simulink library "mssSimulink"  (R2024a)
settings: Solver=ode45  StartTime=0.0  StopTime=10.0  RelTol=1e-3
undefined symbols (not defined in the file): ABC, CN_data, CX_data, CY_data, D, G, Hoerner, K_supply, kt2ms, MA, magnitude, MRB, pathlength, RAO_Amp, RAO_Dir, RAO_Freq, RAO_Phase, RAO_Vel, RAO_yaw_back, RAO_yaw_quant, RAO_yaw_quantization_flag, rho_a, slcm, T_supply, table, vessel, vesselABC
libraries: $bdroot x99, simulink x13
(part 9 of 9)

== system mssSimulink/Environment/Wind/Wind/Wind gust/NORSOK spectrum ==
  Freqs : Inport
  u10 : Inport  Port=2
  5/(3n) (NORSOK parameter) : Constant  Value=5/(3*0.468)
  Constant2 : Constant
  Fcn2 : Fcn  Expr=u^(2/3)
  Fcn3 : Fcn  Expr=(u+1E-4)^(-3/4)
  Fcn4 : Fcn  Expr=u^0.45
  Gain1 : Gain  Gain=172  SaturateOnIntegerOverflow=on  OutDataTypeStr=Inherit: Same as input  ParamDataTypeStr=Inherit: Same as input
  Gain2 : Gain  Gain=1/10  SaturateOnIntegerOverflow=on  OutDataTypeStr=Inherit: Same as input  ParamDataTypeStr=Inherit: Same as input
  Gain3 : Gain  Gain=1/10  SaturateOnIntegerOverflow=on  OutDataTypeStr=Inherit: Same as input  ParamDataTypeStr=Inherit: Same as input
  Gain4 : Gain  Gain=320  SaturateOnIntegerOverflow=on  OutDataTypeStr=Inherit: Same as input  ParamDataTypeStr=Inherit: Same as input
  Math Function3 : Math  Operator=magnitude^2  SignedPower=on
  Math Function4 : Math  Operator=pow  SignedPower=on
  Math Function5 : Math  Operator=pow  SignedPower=on
  Product3 : Product  Inputs=3  SaturateOnIntegerOverflow=on  OutDataTypeStr=Inherit: Same as first input
  Product4 : Product  Inputs=/**  SaturateOnIntegerOverflow=on  OutDataTypeStr=Inherit: Same as first input
  Sum1 : Sum  Inputs=++|  SaturateOnIntegerOverflow=on
  n (NORSOK parameter) : Constant  Value=0.468
  z (height) : Constant  Value=Par_Wind_z
  S : Outport  VectorParamsAs1DForOutWhenUnconnected=off
  wires:
  Freqs/1 -> Gain1/1
  Gain1/1 -> Product3/1
  z (height)/1 -> Gain2/1
  Gain2/1 -> Fcn2/1, Fcn4/1
  Fcn2/1 -> Product3/2
  u10/1 -> Gain3/1
  Gain3/1 -> Fcn3/1, Math Function3/1
  Fcn3/1 -> Product3/3
  Product3/1 -> Math Function4/1  "x"
  n (NORSOK parameter)/1 -> Math Function4/2
  Math Function4/1 -> Sum1/2
  Constant2/1 -> Sum1/1
  Sum1/1 -> Math Function5/1
  Math Function5/1 -> Product4/1
  Fcn4/1 -> Gain4/1
  Math Function3/1 -> Product4/3
  Gain4/1 -> Product4/2
  Product4/1 -> S/1
  5/(3n) (NORSOK parameter)/1 -> Math Function5/2

== system mssSimulink/Environment/Wind/Wind/Wind gust/Phase generator ==
  Trigger : TriggerPort  VariantControl=(inherit)
  Random Number : RandomNumber  Variance=3  Seed=Par_Wind_phase_seed*[1:Par_Wind_nfreq]
  "SSA " : MATLABFcn  MATLABFcn=ssa
  Phase : Outport  VectorParamsAs1DForOutWhenUnconnected=off
  wires:
  Random Number/1 -> "SSA "/1
  "SSA "/1 -> Phase/1

== system mssSimulink/Hydrodynamics/Wave loads (U>0)/Wave loads U = U2/Wave loads for heading1/Wave component loop ==
  number of iterations : Inport
  Psi_r : Inport  Port=2
  Omega : Inport  Port=3
  Phase_tot : Inport  Port=4
  Zeta_a : Inport  Port=5
  U_idx : Inport  Port=6
  "                " : Trigonometry
  Direct Lookup Table (n-D) Beta : LookupNDDirect  NumberOfTableDimensions=1  Table=vessel.headings
  Direct Lookup Table (n-D) Velocity : LookupNDDirect  NumberOfTableDimensions=1  Table=RAO_Vel
  For Iterator : ForIterator  ResetStates=reset  IterationSource=external  IterationVariableDataType=double
  Force RAO tables : Subsystem  mask(RAO table lookup){}
      mask help:
      | Perform 3D table lookup in 6DOF RAO amplitudes and phases, using the relative wave heading psi_r, wave frequency omega and vessel velocity vel as inputs. See documentation of the Motion RAO block or Force RAO block for details. A warning is issued if the input is outside the range spanned by the RAOs.
      |
      | Author: Oyvind N. Smogeli and Thor I. Fossen, 2005-05-03
  Memory1 : Memory  InitialCondition=[0 0 0 0 0 0]'  InheritSampleTime=on
  Memory2 : Memory  InitialCondition=[0 0 0 0 0 0]'  InheritSampleTime=on
  Prelookup1 : PreLookup  BreakpointsData=vessel.headings  OutputSelection=Index only  IndexSearchMethod=Evenly spaced points  BeginIndexSearchUsingPreviousIndexResult=on
  Product1 : Product  SaturateOnIntegerOverflow=on  OutDataTypeStr=Inherit: Same as first input
  Product3 : Product  Inputs=3  SaturateOnIntegerOverflow=on  OutDataTypeStr=Inherit: Same as first input
  Product4 : Product  SaturateOnIntegerOverflow=on  OutDataTypeStr=Inherit: Same as first input
  Selector{2..5} (4 alike) : Selector  IndexOptions=Index vector (port)  Indices=[1 3]  OutputSizes=1
  Sum1 : Sum  Inputs=++|  SaturateOnIntegerOverflow=on
  Sum4 : Sum  Inputs=++|  SaturateOnIntegerOverflow=on
  Sum5 : Sum  Inputs=++|  SaturateOnIntegerOverflow=on
  WD RAO tables : Subsystem  mask(RAO table lookup){}
      mask help:
      | Perform 3D table lookup in 6DOF RAO amplitudes and phases, using the relative wave heading psi_r, wave frequency omega and vessel velocity vel as inputs. See documentation of the Motion RAO block or Force RAO block for details. A warning is issued if the input is outside the range spanned by the RAOs.
      |
      | Author: Oyvind N. Smogeli and Thor I. Fossen, 2005-05-03
  "[-inf inf] to [-pi pi] " : $bdroot/Utilities/Math Operations/[-inf inf] to [-pi pi]
  "[-pi pi] to [0 2pi]" : Subsystem  mask([-inf inf] to [-pi pi]){}
      mask help: Converts an angle in rad to (-pi pi)
  tau_WF : Outport
  tau_WD : Outport  Port=2
  wires:
  Direct Lookup Table (n-D) Velocity/1 -> WD RAO tables/3(U), Force RAO tables/3(U)
  U_idx/1 -> Direct Lookup Table (n-D) Velocity/1
  Direct Lookup Table (n-D) Beta/1 -> WD RAO tables/1(beta), Force RAO tables/1(beta)
  Prelookup1/1 -> Direct Lookup Table (n-D) Beta/1
  "[-inf inf] to [-pi pi] "/1 -> "[-pi pi] to [0 2pi]"/1(x [-pi pi])
  For Iterator/1 -> Selector5/2, Selector4/2, Selector2/2, Selector3/2  "i=1:N"
  Selector2/1 -> WD RAO tables/2(w), Force RAO tables/2(w)  "omega"
  "[-pi pi] to [0 2pi]"/1(0<y<2pi) -> Prelookup1/1
  WD RAO tables/1(amp) -> Product3/1
  Product3/1 -> Sum1/1
  Memory1/1 -> Sum1/2
  Sum1/1 -> tau_WD/1, Memory1/1
  Product4/1 -> Product1/2
  "                "/1 -> Product1/1
  Selector3/1 -> "[-inf inf] to [-pi pi] "/1  "psi_r"
  Selector5/1 -> Sum5/2  "phase"
  Product1/1 -> Sum4/1
  Memory2/1 -> Sum4/2
  Sum4/1 -> tau_WF/1, Memory2/1
  number of iterations/1 -> For Iterator/1
  Omega/1 -> Selector2/1
  Psi_r/1 -> Selector3/1
  Force RAO tables/1(amp) -> Product4/1
  Force RAO tables/2(phase) -> Sum5/1
  Phase_tot/1 -> Selector5/1
  Zeta_a/1 -> Selector4/1
  Sum5/1 -> "                "/1
  Selector4/1 -> Product3/3, Product3/2, Product4/2  "zeta_a"

== system mssSimulink/Hydrodynamics/Wave loads (U>0)/Wave loads U = U2/Wave loads for heading2/Wave component loop ==
  number of iterations : Inport
  Psi_r : Inport  Port=2
  Omega : Inport  Port=3
  Phase_tot : Inport  Port=4
  Zeta_a : Inport  Port=5
  U : Inport  Port=6
  "                " : Trigonometry
  Direct Lookup Table (n-D) : LookupNDDirect  NumberOfTableDimensions=1  Table=vessel.headings
  Direct Lookup Table (n-D)1 : LookupNDDirect  NumberOfTableDimensions=1  Table=RAO_Vel
  For Iterator : ForIterator  ResetStates=reset  IterationSource=external  IterationVariableDataType=double
  Force RAO tables : Subsystem  mask(RAO table lookup){}
      mask help:
      | Perform 3D table lookup in 6DOF RAO amplitudes and phases, using the relative wave heading psi_r, wave frequency omega and vessel velocity vel as inputs. See documentation of the Motion RAO block or Force RAO block for details. A warning is issued if the input is outside the range spanned by the RAOs.
      |
      | Copyright (C) NTNU 2005
      |
      | Author: Oyvind N. Smogeli, 2005-05-03
  Memory1 : Memory  InitialCondition=[0 0 0 0 0 0]'  InheritSampleTime=on
  Memory2 : Memory  InitialCondition=[0 0 0 0 0 0]'  InheritSampleTime=on
  Prelookup : PreLookup  BreakpointsData=vessel.headings  OutputSelection=Index only  IndexSearchMethod=Evenly spaced points  BeginIndexSearchUsingPreviousIndexResult=on
  Product1 : Product  SaturateOnIntegerOverflow=on  OutDataTypeStr=Inherit: Same as first input
  Product3 : Product  Inputs=3  SaturateOnIntegerOverflow=on  OutDataTypeStr=Inherit: Same as first input
  Product4 : Product  SaturateOnIntegerOverflow=on  OutDataTypeStr=Inherit: Same as first input
  Selector{2..5} (4 alike) : Selector  IndexOptions=Index vector (port)  Indices=[1 3]  OutputSizes=1
  Sum1 : Sum  Inputs=++|  SaturateOnIntegerOverflow=on
  Sum4 : Sum  Inputs=++|  SaturateOnIntegerOverflow=on
  Sum5 : Sum  Inputs=++|  SaturateOnIntegerOverflow=on
  WD RAO tables : Subsystem  mask(RAO table lookup){}
      mask help:
      | Perform 3D table lookup in 6DOF RAO amplitudes and phases, using the relative wave heading psi_r, wave frequency omega and vessel velocity vel as inputs. See documentation of the Motion RAO block or Force RAO block for details. A warning is issued if the input is outside the range spanned by the RAOs.
      |
      | Copyright (C) NTNU 2005
      |
      | Author: Oyvind N. Smogeli, 2005-05-03
  "[-inf inf] to [-pi pi] " : $bdroot/Utilities/Math Operations/[-inf inf] to [-pi pi]
  "[-pi pi] to [0 2pi]" : Subsystem  mask([-inf inf] to [-pi pi]){}
      mask help: Converts an angle in rad to (-pi pi)
  tau_WF : Outport
  tau_WD : Outport  Port=2
  wires:
  Direct Lookup Table (n-D)1/1 -> WD RAO tables/3(U), Force RAO tables/3(U)
  Direct Lookup Table (n-D)/1 -> WD RAO tables/1(beta), Force RAO tables/1(beta)
  Prelookup/1 -> Direct Lookup Table (n-D)/1
  "[-inf inf] to [-pi pi] "/1 -> "[-pi pi] to [0 2pi]"/1(x [-pi pi])
  For Iterator/1 -> Selector5/2, Selector4/2, Selector2/2, Selector3/2  "i=1:N"
  Selector2/1 -> WD RAO tables/2(w), Force RAO tables/2(w)  "omega"
  "[-pi pi] to [0 2pi]"/1(0<y<2pi) -> Prelookup/1
  WD RAO tables/1(amp) -> Product3/1
  Product3/1 -> Sum1/1
  Memory1/1 -> Sum1/2
  Sum1/1 -> tau_WD/1, Memory1/1
  Product4/1 -> Product1/2
  "                "/1 -> Product1/1
  Selector3/1 -> "[-inf inf] to [-pi pi] "/1  "psi_r"
  Selector5/1 -> Sum5/2  "phase"
  Product1/1 -> Sum4/1
  Memory2/1 -> Sum4/2
  Sum4/1 -> tau_WF/1, Memory2/1
  number of iterations/1 -> For Iterator/1
  Omega/1 -> Selector2/1
  Psi_r/1 -> Selector3/1
  U/1 -> Direct Lookup Table (n-D)1/1
  Force RAO tables/1(amp) -> Product4/1
  Force RAO tables/2(phase) -> Sum5/1
  Phase_tot/1 -> Selector5/1
  Zeta_a/1 -> Selector4/1
  Sum5/1 -> "                "/1
  Selector4/1 -> Product3/3, Product3/2, Product4/2  "zeta_a"

== system mssSimulink/Modelling/Kinetics /Support/6 DOF Coriolis forces/3x3 cross product ==
  a : Inport
  b : Inport  Port=2
  Product : Product  InputSameDT=on  SaturateOnIntegerOverflow=on  OutDataTypeStr=Inherit: Same as first input
  Product1 : Product  InputSameDT=on  SaturateOnIntegerOverflow=on  OutDataTypeStr=Inherit: Same as first input
  Selector : Selector  InputPortWidth=3  IndexOptions=Index vector (dialog)  Indices=[2 3 1]  OutputSizes=1
  Selector1 : Selector  InputPortWidth=3  IndexOptions=Index vector (dialog)  Indices=[3 1 2]  OutputSizes=1
  Selector2 : Selector  InputPortWidth=3  IndexOptions=Index vector (dialog)  Indices=[2 3 1]  OutputSizes=1
  Selector3 : Selector  InputPortWidth=3  IndexOptions=Index vector (dialog)  Indices=[3 1 2]  OutputSizes=1
  Sum : Sum  Inputs=+|-  InputSameDT=on  SaturateOnIntegerOverflow=on  OutDataTypeStr=Inherit: Same as first input
  c : Outport  InitialOutput=0  VectorParamsAs1DForOutWhenUnconnected=off
  wires:
  Sum/1 -> c/1
  b/1 -> Selector1/1, Selector2/1
  Selector/1 -> Product/1
  a/1 -> Selector/1, Selector3/1
  Product/1 -> Sum/1
  Selector1/1 -> Product/2
  Product1/1 -> Sum/2
  Selector2/1 -> Product1/2
  Selector3/1 -> Product1/1

== system mssSimulink/Modelling/Kinetics /Support/6 DOF Coriolis forces/3x3 cross product1 ==
  a : Inport
  b : Inport  Port=2
  Product : Product  InputSameDT=on  SaturateOnIntegerOverflow=on  OutDataTypeStr=Inherit: Same as first input
  Product1 : Product  InputSameDT=on  SaturateOnIntegerOverflow=on  OutDataTypeStr=Inherit: Same as first input
  Selector : Selector  InputPortWidth=3  IndexOptions=Index vector (dialog)  Indices=[2 3 1]  OutputSizes=1
  Selector1 : Selector  InputPortWidth=3  IndexOptions=Index vector (dialog)  Indices=[3 1 2]  OutputSizes=1
  Selector2 : Selector  InputPortWidth=3  IndexOptions=Index vector (dialog)  Indices=[2 3 1]  OutputSizes=1
  Selector3 : Selector  InputPortWidth=3  IndexOptions=Index vector (dialog)  Indices=[3 1 2]  OutputSizes=1
  Sum : Sum  Inputs=+|-  InputSameDT=on  SaturateOnIntegerOverflow=on  OutDataTypeStr=Inherit: Same as first input
  c : Outport  InitialOutput=0  VectorParamsAs1DForOutWhenUnconnected=off
  wires:
  Sum/1 -> c/1
  b/1 -> Selector1/1, Selector2/1
  Selector/1 -> Product/1
  a/1 -> Selector/1, Selector3/1
  Product/1 -> Sum/1
  Selector1/1 -> Product/2
  Product1/1 -> Sum/2
  Selector2/1 -> Product1/2
  Selector3/1 -> Product1/1

== system mssSimulink/Modelling/Kinetics /Support/6 DOF Coriolis forces/3x3 cross product2 ==
  a : Inport
  b : Inport  Port=2
  Product : Product  InputSameDT=on  SaturateOnIntegerOverflow=on  OutDataTypeStr=Inherit: Same as first input
  Product1 : Product  InputSameDT=on  SaturateOnIntegerOverflow=on  OutDataTypeStr=Inherit: Same as first input
  Selector : Selector  InputPortWidth=3  IndexOptions=Index vector (dialog)  Indices=[2 3 1]  OutputSizes=1
  Selector1 : Selector  InputPortWidth=3  IndexOptions=Index vector (dialog)  Indices=[3 1 2]  OutputSizes=1
  Selector2 : Selector  InputPortWidth=3  IndexOptions=Index vector (dialog)  Indices=[2 3 1]  OutputSizes=1
  Selector3 : Selector  InputPortWidth=3  IndexOptions=Index vector (dialog)  Indices=[3 1 2]  OutputSizes=1
  Sum : Sum  Inputs=+|-  InputSameDT=on  SaturateOnIntegerOverflow=on  OutDataTypeStr=Inherit: Same as first input
  c : Outport  InitialOutput=0  VectorParamsAs1DForOutWhenUnconnected=off
  wires:
  Sum/1 -> c/1
  b/1 -> Selector1/1, Selector2/1
  Selector/1 -> Product/1
  a/1 -> Selector/1, Selector3/1
  Product/1 -> Sum/1
  Selector1/1 -> Product/2
  Product1/1 -> Sum/2
  Selector2/1 -> Product1/2
  Selector3/1 -> Product1/1

== system mssSimulink/Hydrodynamics/Wave loads (U>0)/Wave loads U = U2/Wave loads for heading1/Wave component loop/Force RAO tables ==
  beta : Inport
  w : Inport  Port=2
  U : Inport  Port=3
  Lookup Table (n-D) Amp1 : Lookup_n-D  NumberOfTableDimensions=3  BreakpointsForDimension1=ForceRAO_Freq  BreakpointsForDimension2=vessel.headings  BreakpointsForDimension3=RAO_Vel  IndexSearchMethod=Linear search  BeginIndexSearchUsingPreviousIndexResult=on  Table=ForceRAO_Amp{1}  ExtrapMethod=Clip  DiagnosticForOutOfRangeInput=Warning  InternalRulePriority=Speed  RndMeth=Simplest
      settings: InputPortMap=u0,u1,u2
  Lookup Table (n-D) Amp2 : Lookup_n-D  NumberOfTableDimensions=3  BreakpointsForDimension1=ForceRAO_Freq  BreakpointsForDimension2=vessel.headings  BreakpointsForDimension3=RAO_Vel  IndexSearchMethod=Linear search  BeginIndexSearchUsingPreviousIndexResult=on  Table=ForceRAO_Amp{2}  ExtrapMethod=Clip  DiagnosticForOutOfRangeInput=Warning  InternalRulePriority=Speed  RndMeth=Simplest
      settings: InputPortMap=u0,u1,u2
  Lookup Table (n-D) Amp3 : Lookup_n-D  NumberOfTableDimensions=3  BreakpointsForDimension1=ForceRAO_Freq  BreakpointsForDimension2=vessel.headings  BreakpointsForDimension3=RAO_Vel  IndexSearchMethod=Linear search  BeginIndexSearchUsingPreviousIndexResult=on  Table=ForceRAO_Amp{3}  ExtrapMethod=Clip  DiagnosticForOutOfRangeInput=Warning  InternalRulePriority=Speed  RndMeth=Simplest
      settings: InputPortMap=u0,u1,u2
  Lookup Table (n-D) Amp4 : Lookup_n-D  NumberOfTableDimensions=3  BreakpointsForDimension1=ForceRAO_Freq  BreakpointsForDimension2=vessel.headings  BreakpointsForDimension3=RAO_Vel  IndexSearchMethod=Linear search  BeginIndexSearchUsingPreviousIndexResult=on  Table=ForceRAO_Amp{4}  ExtrapMethod=Clip  DiagnosticForOutOfRangeInput=Warning  InternalRulePriority=Speed  RndMeth=Simplest
      settings: InputPortMap=u0,u1,u2
  Lookup Table (n-D) Amp5 : Lookup_n-D  NumberOfTableDimensions=3  BreakpointsForDimension1=ForceRAO_Freq  BreakpointsForDimension2=vessel.headings  BreakpointsForDimension3=RAO_Vel  IndexSearchMethod=Linear search  BeginIndexSearchUsingPreviousIndexResult=on  Table=ForceRAO_Amp{5}  ExtrapMethod=Clip  DiagnosticForOutOfRangeInput=Warning  InternalRulePriority=Speed  RndMeth=Simplest
      settings: InputPortMap=u0,u1,u2
  Lookup Table (n-D) Amp6 : Lookup_n-D  NumberOfTableDimensions=3  BreakpointsForDimension1=ForceRAO_Freq  BreakpointsForDimension2=vessel.headings  BreakpointsForDimension3=RAO_Vel  IndexSearchMethod=Linear search  BeginIndexSearchUsingPreviousIndexResult=on  Table=ForceRAO_Amp{6}  ExtrapMethod=Clip  DiagnosticForOutOfRangeInput=Warning  InternalRulePriority=Speed  RndMeth=Simplest
      settings: InputPortMap=u0,u1,u2
  Lookup Table (n-D) Phase : Lookup_n-D  NumberOfTableDimensions=3  BreakpointsForDimension1=ForceRAO_Freq  BreakpointsForDimension2=vessel.headings  BreakpointsForDimension3=RAO_Vel  IndexSearchMethod=Linear search  BeginIndexSearchUsingPreviousIndexResult=on  Table=ForceRAO_Phase{3}  ExtrapMethod=Clip  DiagnosticForOutOfRangeInput=Warning  InternalRulePriority=Speed  RndMeth=Simplest
      settings: InputPortMap=u0,u1,u2
  Lookup Table (n-D) Phase1 : Lookup_n-D  NumberOfTableDimensions=3  BreakpointsForDimension1=ForceRAO_Freq  BreakpointsForDimension2=vessel.headings  BreakpointsForDimension3=RAO_Vel  IndexSearchMethod=Linear search  BeginIndexSearchUsingPreviousIndexResult=on  Table=ForceRAO_Phase{1}  ExtrapMethod=Clip  DiagnosticForOutOfRangeInput=Warning  InternalRulePriority=Speed  RndMeth=Simplest
      settings: InputPortMap=u0,u1,u2
  Lookup Table (n-D) Phase2 : Lookup_n-D  NumberOfTableDimensions=3  BreakpointsForDimension1=ForceRAO_Freq  BreakpointsForDimension2=vessel.headings  BreakpointsForDimension3=RAO_Vel  IndexSearchMethod=Linear search  BeginIndexSearchUsingPreviousIndexResult=on  Table=ForceRAO_Phase{2}  ExtrapMethod=Clip  DiagnosticForOutOfRangeInput=Warning  InternalRulePriority=Speed  RndMeth=Simplest
      settings: InputPortMap=u0,u1,u2
  Lookup Table (n-D) Phase4 : Lookup_n-D  NumberOfTableDimensions=3  BreakpointsForDimension1=ForceRAO_Freq  BreakpointsForDimension2=vessel.headings  BreakpointsForDimension3=RAO_Vel  IndexSearchMethod=Linear search  BeginIndexSearchUsingPreviousIndexResult=on  Table=ForceRAO_Phase{4}  ExtrapMethod=Clip  DiagnosticForOutOfRangeInput=Warning  InternalRulePriority=Speed  RndMeth=Simplest
      settings: InputPortMap=u0,u1,u2
  Lookup Table (n-D) Phase5 : Lookup_n-D  NumberOfTableDimensions=3  BreakpointsForDimension1=ForceRAO_Freq  BreakpointsForDimension2=vessel.headings  BreakpointsForDimension3=RAO_Vel  IndexSearchMethod=Linear search  BeginIndexSearchUsingPreviousIndexResult=on  Table=ForceRAO_Phase{5}  ExtrapMethod=Clip  DiagnosticForOutOfRangeInput=Warning  InternalRulePriority=Speed  RndMeth=Simplest
      settings: InputPortMap=u0,u1,u2
  Lookup Table (n-D) Phase6 : Lookup_n-D  NumberOfTableDimensions=3  BreakpointsForDimension1=ForceRAO_Freq  BreakpointsForDimension2=vessel.headings  BreakpointsForDimension3=RAO_Vel  IndexSearchMethod=Linear search  BeginIndexSearchUsingPreviousIndexResult=on  Table=ForceRAO_Phase{6}  ExtrapMethod=Clip  DiagnosticForOutOfRangeInput=Warning  InternalRulePriority=Speed  RndMeth=Simplest
      settings: InputPortMap=u0,u1,u2
  Mux1 : Mux  Inputs=6
  Mux2 : Mux  Inputs=6
  amp : Outport
  phase : Outport  Port=2
  wires:
  w/1 -> Lookup Table (n-D) Amp1/1, Lookup Table (n-D) Amp2/1, Lookup Table (n-D) Amp3/1, Lookup Table (n-D) Amp4/1, Lookup Table (n-D) Amp5/1, Lookup Table (n-D) Amp6/1, Lookup Table (n-D) Phase1/1, Lookup Table (n-D) Phase2/1, Lookup Table (n-D) Phase/1, Lookup Table (n-D) Phase4/1, Lookup Table (n-D) Phase6/1, Lookup Table (n-D) Phase5/1
  Lookup Table (n-D) Phase5/1 -> Mux2/5
  Lookup Table (n-D) Phase/1 -> Mux2/3
  Lookup Table (n-D) Phase1/1 -> Mux2/1
  beta/1 -> Lookup Table (n-D) Amp1/2, Lookup Table (n-D) Amp2/2, Lookup Table (n-D) Amp3/2, Lookup Table (n-D) Amp4/2, Lookup Table (n-D) Amp5/2, Lookup Table (n-D) Amp6/2, Lookup Table (n-D) Phase1/2, Lookup Table (n-D) Phase2/2, Lookup Table (n-D) Phase/2, Lookup Table (n-D) Phase4/2, Lookup Table (n-D) Phase6/2, Lookup Table (n-D) Phase5/2
  Lookup Table (n-D) Phase4/1 -> Mux2/4
  Lookup Table (n-D) Phase2/1 -> Mux2/2
  Lookup Table (n-D) Phase6/1 -> Mux2/6
  Lookup Table (n-D) Amp4/1 -> Mux1/4
  U/1 -> Lookup Table (n-D) Amp1/3, Lookup Table (n-D) Amp2/3, Lookup Table (n-D) Amp3/3, Lookup Table (n-D) Amp4/3, Lookup Table (n-D) Amp5/3, Lookup Table (n-D) Amp6/3, Lookup Table (n-D) Phase1/3, Lookup Table (n-D) Phase2/3, Lookup Table (n-D) Phase/3, Lookup Table (n-D) Phase4/3, Lookup Table (n-D) Phase6/3, Lookup Table (n-D) Phase5/3
  Lookup Table (n-D) Amp1/1 -> Mux1/1
  Lookup Table (n-D) Amp3/1 -> Mux1/3
  Lookup Table (n-D) Amp5/1 -> Mux1/5
  Lookup Table (n-D) Amp2/1 -> Mux1/2
  Lookup Table (n-D) Amp6/1 -> Mux1/6
  Mux2/1 -> phase/1
  Mux1/1 -> amp/1

== system mssSimulink/Hydrodynamics/Wave loads (U>0)/Wave loads U = U2/Wave loads for heading1/Wave component loop/WD RAO tables ==
  beta : Inport
  w : Inport  Port=2
  U : Inport  Port=3
  Constant : Constant  Value=0
  Lookup Table (n-D) Wavedrift 1 : Lookup_n-D  NumberOfTableDimensions=3  BreakpointsForDimension1=WD_Freq  BreakpointsForDimension2=vessel.headings  BreakpointsForDimension3=RAO_Vel  IndexSearchMethod=Linear search  BeginIndexSearchUsingPreviousIndexResult=on  Table=WD_Amp{1}  ExtrapMethod=Clip  DiagnosticForOutOfRangeInput=Warning  InternalRulePriority=Speed  RndMeth=Simplest
      settings: InputPortMap=u0,u1,u2
  Lookup Table (n-D) Wavedrift 2 : Lookup_n-D  NumberOfTableDimensions=3  BreakpointsForDimension1=WD_Freq  BreakpointsForDimension2=vessel.headings  BreakpointsForDimension3=RAO_Vel  IndexSearchMethod=Linear search  BeginIndexSearchUsingPreviousIndexResult=on  Table=WD_Amp{2}  ExtrapMethod=Clip  DiagnosticForOutOfRangeInput=Warning  InternalRulePriority=Speed  RndMeth=Simplest
      settings: InputPortMap=u0,u1,u2
  Lookup Table (n-D) Wavedrift 3 : Lookup_n-D  NumberOfTableDimensions=3  BreakpointsForDimension1=WD_Freq  BreakpointsForDimension2=vessel.headings  BreakpointsForDimension3=RAO_Vel  IndexSearchMethod=Linear search  BeginIndexSearchUsingPreviousIndexResult=on  Table=WD_Amp{3}  ExtrapMethod=Clip  DiagnosticForOutOfRangeInput=Warning  InternalRulePriority=Speed  RndMeth=Simplest
      settings: InputPortMap=u0,u1,u2
  Mux1 : Mux  Inputs=6
  amp : Outport
  wires:
  w/1 -> Lookup Table (n-D) Wavedrift 1/1, Lookup Table (n-D) Wavedrift 3/1, Lookup Table (n-D) Wavedrift 2/1
  Constant/1 -> Mux1/5, Mux1/4, Mux1/3
  beta/1 -> Lookup Table (n-D) Wavedrift 1/2, Lookup Table (n-D) Wavedrift 3/2, Lookup Table (n-D) Wavedrift 2/2
  U/1 -> Lookup Table (n-D) Wavedrift 1/3, Lookup Table (n-D) Wavedrift 3/3, Lookup Table (n-D) Wavedrift 2/3
  Lookup Table (n-D) Wavedrift 1/1 -> Mux1/1
  Lookup Table (n-D) Wavedrift 2/1 -> Mux1/2
  Lookup Table (n-D) Wavedrift 3/1 -> Mux1/6
  Mux1/1 -> amp/1

== system mssSimulink/Hydrodynamics/Wave loads (U>0)/Wave loads U = U2/Wave loads for heading1/Wave component loop/[-pi pi] to [0 2pi] ==
  note: x
  x [-pi pi] : Inport
  Constant : Constant  Value=2*pi
  Constant1 : Constant  Value=0
  Sign : Signum
  Sum : Sum  Inputs=|++  SaturateOnIntegerOverflow=on
  Switch : Switch  SaturateOnIntegerOverflow=off  InputSameDT=off
  0<y<2pi : Outport
  wires:
  Constant1/1 -> Switch/1
  Constant/1 -> Switch/3
  Sign/1 -> Switch/2
  Sum/1 -> 0<y<2pi/1
  Switch/1 -> Sum/1
  x [-pi pi]/1 -> Sum/2, Sign/1

== system mssSimulink/Hydrodynamics/Wave loads (U>0)/Wave loads U = U2/Wave loads for heading2/Wave component loop/Force RAO tables ==
  beta : Inport
  w : Inport  Port=2
  U : Inport  Port=3
  Lookup Table (n-D) Amp1 : Lookup_n-D  NumberOfTableDimensions=3  BreakpointsForDimension1=ForceRAO_Freq  BreakpointsForDimension2=vessel.headings  BreakpointsForDimension3=RAO_Vel  IndexSearchMethod=Linear search  BeginIndexSearchUsingPreviousIndexResult=on  Table=ForceRAO_Amp{1}  ExtrapMethod=Clip  DiagnosticForOutOfRangeInput=Warning  InternalRulePriority=Speed  RndMeth=Simplest
      settings: InputPortMap=u0,u1,u2
  Lookup Table (n-D) Amp2 : Lookup_n-D  NumberOfTableDimensions=3  BreakpointsForDimension1=ForceRAO_Freq  BreakpointsForDimension2=vessel.headings  BreakpointsForDimension3=RAO_Vel  IndexSearchMethod=Linear search  BeginIndexSearchUsingPreviousIndexResult=on  Table=ForceRAO_Amp{2}  ExtrapMethod=Clip  DiagnosticForOutOfRangeInput=Warning  InternalRulePriority=Speed  RndMeth=Simplest
      settings: InputPortMap=u0,u1,u2
  Lookup Table (n-D) Amp3 : Lookup_n-D  NumberOfTableDimensions=3  BreakpointsForDimension1=ForceRAO_Freq  BreakpointsForDimension2=vessel.headings  BreakpointsForDimension3=RAO_Vel  IndexSearchMethod=Linear search  BeginIndexSearchUsingPreviousIndexResult=on  Table=ForceRAO_Amp{3}  ExtrapMethod=Clip  DiagnosticForOutOfRangeInput=Warning  InternalRulePriority=Speed  RndMeth=Simplest
      settings: InputPortMap=u0,u1,u2
  Lookup Table (n-D) Amp4 : Lookup_n-D  NumberOfTableDimensions=3  BreakpointsForDimension1=ForceRAO_Freq  BreakpointsForDimension2=vessel.headings  BreakpointsForDimension3=RAO_Vel  IndexSearchMethod=Linear search  BeginIndexSearchUsingPreviousIndexResult=on  Table=ForceRAO_Amp{4}  ExtrapMethod=Clip  DiagnosticForOutOfRangeInput=Warning  InternalRulePriority=Speed  RndMeth=Simplest
      settings: InputPortMap=u0,u1,u2
  Lookup Table (n-D) Amp5 : Lookup_n-D  NumberOfTableDimensions=3  BreakpointsForDimension1=ForceRAO_Freq  BreakpointsForDimension2=vessel.headings  BreakpointsForDimension3=RAO_Vel  IndexSearchMethod=Linear search  BeginIndexSearchUsingPreviousIndexResult=on  Table=ForceRAO_Amp{5}  ExtrapMethod=Clip  DiagnosticForOutOfRangeInput=Warning  InternalRulePriority=Speed  RndMeth=Simplest
      settings: InputPortMap=u0,u1,u2
  Lookup Table (n-D) Amp6 : Lookup_n-D  NumberOfTableDimensions=3  BreakpointsForDimension1=ForceRAO_Freq  BreakpointsForDimension2=vessel.headings  BreakpointsForDimension3=RAO_Vel  IndexSearchMethod=Linear search  BeginIndexSearchUsingPreviousIndexResult=on  Table=ForceRAO_Amp{6}  ExtrapMethod=Clip  DiagnosticForOutOfRangeInput=Warning  InternalRulePriority=Speed  RndMeth=Simplest
      settings: InputPortMap=u0,u1,u2
  Lookup Table (n-D) Phase : Lookup_n-D  NumberOfTableDimensions=3  BreakpointsForDimension1=ForceRAO_Freq  BreakpointsForDimension2=vessel.headings  BreakpointsForDimension3=RAO_Vel  IndexSearchMethod=Linear search  BeginIndexSearchUsingPreviousIndexResult=on  Table=ForceRAO_Phase{3}  ExtrapMethod=Clip  DiagnosticForOutOfRangeInput=Warning  InternalRulePriority=Speed  RndMeth=Simplest
      settings: InputPortMap=u0,u1,u2
  Lookup Table (n-D) Phase1 : Lookup_n-D  NumberOfTableDimensions=3  BreakpointsForDimension1=ForceRAO_Freq  BreakpointsForDimension2=vessel.headings  BreakpointsForDimension3=RAO_Vel  IndexSearchMethod=Linear search  BeginIndexSearchUsingPreviousIndexResult=on  Table=ForceRAO_Phase{1}  ExtrapMethod=Clip  DiagnosticForOutOfRangeInput=Warning  InternalRulePriority=Speed  RndMeth=Simplest
      settings: InputPortMap=u0,u1,u2
  Lookup Table (n-D) Phase2 : Lookup_n-D  NumberOfTableDimensions=3  BreakpointsForDimension1=ForceRAO_Freq  BreakpointsForDimension2=vessel.headings  BreakpointsForDimension3=RAO_Vel  IndexSearchMethod=Linear search  BeginIndexSearchUsingPreviousIndexResult=on  Table=ForceRAO_Phase{2}  ExtrapMethod=Clip  DiagnosticForOutOfRangeInput=Warning  InternalRulePriority=Speed  RndMeth=Simplest
      settings: InputPortMap=u0,u1,u2
  Lookup Table (n-D) Phase4 : Lookup_n-D  NumberOfTableDimensions=3  BreakpointsForDimension1=ForceRAO_Freq  BreakpointsForDimension2=vessel.headings  BreakpointsForDimension3=RAO_Vel  IndexSearchMethod=Linear search  BeginIndexSearchUsingPreviousIndexResult=on  Table=ForceRAO_Phase{4}  ExtrapMethod=Clip  DiagnosticForOutOfRangeInput=Warning  InternalRulePriority=Speed  RndMeth=Simplest
      settings: InputPortMap=u0,u1,u2
  Lookup Table (n-D) Phase5 : Lookup_n-D  NumberOfTableDimensions=3  BreakpointsForDimension1=ForceRAO_Freq  BreakpointsForDimension2=vessel.headings  BreakpointsForDimension3=RAO_Vel  IndexSearchMethod=Linear search  BeginIndexSearchUsingPreviousIndexResult=on  Table=ForceRAO_Phase{5}  ExtrapMethod=Clip  DiagnosticForOutOfRangeInput=Warning  InternalRulePriority=Speed  RndMeth=Simplest
      settings: InputPortMap=u0,u1,u2
  Lookup Table (n-D) Phase6 : Lookup_n-D  NumberOfTableDimensions=3  BreakpointsForDimension1=ForceRAO_Freq  BreakpointsForDimension2=vessel.headings  BreakpointsForDimension3=RAO_Vel  IndexSearchMethod=Linear search  BeginIndexSearchUsingPreviousIndexResult=on  Table=ForceRAO_Phase{6}  ExtrapMethod=Clip  DiagnosticForOutOfRangeInput=Warning  InternalRulePriority=Speed  RndMeth=Simplest
      settings: InputPortMap=u0,u1,u2
  Mux1 : Mux  Inputs=6
  Mux2 : Mux  Inputs=6
  amp : Outport
  phase : Outport  Port=2
  wires:
  w/1 -> Lookup Table (n-D) Amp1/1, Lookup Table (n-D) Amp2/1, Lookup Table (n-D) Amp3/1, Lookup Table (n-D) Amp4/1, Lookup Table (n-D) Amp5/1, Lookup Table (n-D) Amp6/1, Lookup Table (n-D) Phase1/1, Lookup Table (n-D) Phase2/1, Lookup Table (n-D) Phase/1, Lookup Table (n-D) Phase4/1, Lookup Table (n-D) Phase6/1, Lookup Table (n-D) Phase5/1
  Lookup Table (n-D) Phase5/1 -> Mux2/5
  Lookup Table (n-D) Phase/1 -> Mux2/3
  Lookup Table (n-D) Phase1/1 -> Mux2/1
  beta/1 -> Lookup Table (n-D) Amp1/2, Lookup Table (n-D) Amp2/2, Lookup Table (n-D) Amp3/2, Lookup Table (n-D) Amp4/2, Lookup Table (n-D) Amp5/2, Lookup Table (n-D) Amp6/2, Lookup Table (n-D) Phase1/2, Lookup Table (n-D) Phase2/2, Lookup Table (n-D) Phase/2, Lookup Table (n-D) Phase4/2, Lookup Table (n-D) Phase6/2, Lookup Table (n-D) Phase5/2
  Lookup Table (n-D) Phase4/1 -> Mux2/4
  Lookup Table (n-D) Phase2/1 -> Mux2/2
  Lookup Table (n-D) Phase6/1 -> Mux2/6
  Lookup Table (n-D) Amp4/1 -> Mux1/4
  U/1 -> Lookup Table (n-D) Amp1/3, Lookup Table (n-D) Amp2/3, Lookup Table (n-D) Amp3/3, Lookup Table (n-D) Amp4/3, Lookup Table (n-D) Amp5/3, Lookup Table (n-D) Amp6/3, Lookup Table (n-D) Phase1/3, Lookup Table (n-D) Phase2/3, Lookup Table (n-D) Phase/3, Lookup Table (n-D) Phase4/3, Lookup Table (n-D) Phase6/3, Lookup Table (n-D) Phase5/3
  Lookup Table (n-D) Amp1/1 -> Mux1/1
  Lookup Table (n-D) Amp3/1 -> Mux1/3
  Lookup Table (n-D) Amp5/1 -> Mux1/5
  Lookup Table (n-D) Amp2/1 -> Mux1/2
  Lookup Table (n-D) Amp6/1 -> Mux1/6
  Mux2/1 -> phase/1
  Mux1/1 -> amp/1

== system mssSimulink/Hydrodynamics/Wave loads (U>0)/Wave loads U = U2/Wave loads for heading2/Wave component loop/WD RAO tables ==
  beta : Inport
  w : Inport  Port=2
  U : Inport  Port=3
  Constant : Constant  Value=0
  Lookup Table (n-D) Wavedrift 1 : Lookup_n-D  NumberOfTableDimensions=3  BreakpointsForDimension1=WD_Freq  BreakpointsForDimension2=vessel.headings  BreakpointsForDimension3=RAO_Vel  IndexSearchMethod=Linear search  BeginIndexSearchUsingPreviousIndexResult=on  Table=WD_Amp{1}  ExtrapMethod=Clip  DiagnosticForOutOfRangeInput=Warning  InternalRulePriority=Speed  RndMeth=Simplest
      settings: InputPortMap=u0,u1,u2
  Lookup Table (n-D) Wavedrift 2 : Lookup_n-D  NumberOfTableDimensions=3  BreakpointsForDimension1=WD_Freq  BreakpointsForDimension2=vessel.headings  BreakpointsForDimension3=RAO_Vel  IndexSearchMethod=Linear search  BeginIndexSearchUsingPreviousIndexResult=on  Table=WD_Amp{2}  ExtrapMethod=Clip  DiagnosticForOutOfRangeInput=Warning  InternalRulePriority=Speed  RndMeth=Simplest
      settings: InputPortMap=u0,u1,u2
  Lookup Table (n-D) Wavedrift 3 : Lookup_n-D  NumberOfTableDimensions=3  BreakpointsForDimension1=WD_Freq  BreakpointsForDimension2=vessel.headings  BreakpointsForDimension3=RAO_Vel  IndexSearchMethod=Linear search  BeginIndexSearchUsingPreviousIndexResult=on  Table=WD_Amp{3}  ExtrapMethod=Clip  DiagnosticForOutOfRangeInput=Warning  InternalRulePriority=Speed  RndMeth=Simplest
      settings: InputPortMap=u0,u1,u2
  Mux1 : Mux  Inputs=6
  amp : Outport
  wires:
  w/1 -> Lookup Table (n-D) Wavedrift 1/1, Lookup Table (n-D) Wavedrift 3/1, Lookup Table (n-D) Wavedrift 2/1
  Constant/1 -> Mux1/5, Mux1/4, Mux1/3
  beta/1 -> Lookup Table (n-D) Wavedrift 1/2, Lookup Table (n-D) Wavedrift 3/2, Lookup Table (n-D) Wavedrift 2/2
  U/1 -> Lookup Table (n-D) Wavedrift 1/3, Lookup Table (n-D) Wavedrift 3/3, Lookup Table (n-D) Wavedrift 2/3
  Lookup Table (n-D) Wavedrift 1/1 -> Mux1/1
  Lookup Table (n-D) Wavedrift 2/1 -> Mux1/2
  Lookup Table (n-D) Wavedrift 3/1 -> Mux1/6
  Mux1/1 -> amp/1

== system mssSimulink/Hydrodynamics/Wave loads (U>0)/Wave loads U = U2/Wave loads for heading2/Wave component loop/[-pi pi] to [0 2pi] ==
  note: x
  x [-pi pi] : Inport
  Constant : Constant  Value=2*pi
  Constant1 : Constant  Value=0
  Sign : Signum
  Sum : Sum  Inputs=|++  SaturateOnIntegerOverflow=on
  Switch : Switch  SaturateOnIntegerOverflow=off  InputSameDT=off
  0<y<2pi : Outport
  wires:
  Constant1/1 -> Switch/1
  Constant/1 -> Switch/3
  Sign/1 -> Switch/2
  Sum/1 -> 0<y<2pi/1
  Switch/1 -> Sum/1
  x [-pi pi]/1 -> Sum/2, Sign/1

== matlab function mssSimulink/Guidance/ALOS guidance law for heading autopilot ==
  settings: updateMethod=DISCRETE
  data: x input; y input; psi_ref output; Delta_h input; gamma_h input; R_switch input; xdata input; ydata input; h input
function psi_ref = fcn(x,y,Delta_h,gamma_h,R_switch,xdata,ydata,h)

% waypoints
wpt.pos.x = xdata;
wpt.pos.y = ydata;

% ILOS guidance law
psi_ref = ALOSpsi(x,y,Delta_h,gamma_h,h,R_switch,wpt);
          ALOSpsi(x,y,Delta_h,gamma_h,h,R_switch,wpt);

end

== matlab function mssSimulink/Navigation/Estimators/Discerte-time EKF for SOG and COG/Five-state EKF for North-East positions ==
  settings: updateMethod=DISCRETE
  data: position1 input; x_hat output; position2 input; h_samp input; Qd input; Rd input; alpha_1 input; alpha_2 input
function x_hat = EKF_5states(position1,position2,h_samp,Qd,Rd,alpha_1,alpha_2) 
% This function estimates the Speed Over Ground (SOG), Course Over Ground 
% (COG), and course rate from positions measurements (x, y) expressed in
% NED using the 5-state discrete-time extended Kalamn filter (EKF) of 
% Fossen and Fossen (2021). The states estimated include positions (x, y), 
% SOG (U), COG (chi), and course rate (omega_chi) in the NED coordinate system.
%
% Inputs:
%   position1 - x position measurement in meters.
%   position2 - y position measurement in meters.
%   h_samp    - Sampling time in seconds.
%   Qd        - Process noise covariance matrix (5x5).
%   Rd        - Measurement noise covariance matrix (2x2).
%   alpha_1   - Singer constant, SOG.
%   alpha_2   - Singer constant, COG.
%
% Output:
%   x_hat     - Estimated state vector [x, y, U, chi, omega_chi], where:
%               x, y     - Estimated positions in meters.
%               U        - Estimated Speed Over Ground (SOG) in m/s.
%               chi      - Estimated Course Over Ground (COG) in radians.
%               omega_chi- Estimated rate of change of COG in rad/s.
%
% Example usage:
%   Qd = diag([0.1, 0.1, 0.01, 0.01, 0.001]);
%   Rd = diag([0.05, 0.05]);
%   x_hat = EKF_5states(x, y, 0.1, Qd, Rd, 0.00001, 0.00001);
%
% Refernces:
%   S. Fossen and T. I. Fossen (2021). Five-state Extended Kalman Filter 
%   for Estimation of Speed Over Ground (SOG), Course Over Ground (COG) 
%   and Course Rate of Unmanned Surface Vehicles (USVs): Experimental 
%   Results. Sensors 21(23).

persistent x_prd;
persistent P_prd;

if isempty(x_prd)
   x_prd = [ position1 position2 0 0 0 ]';
   P_prd = eye(5);  
end

Cd  = [1 0 0 0 0
       0 1 0 0 0 ];
Ed = h_samp * [ 0 0; 0 0; 1 0; 0 0; 0 1 ];

y  = [ position1        % y1 = x^n    
       position2 ];     % y2 = y^n    

K = P_prd * Cd' / ( Cd * P_prd * Cd' + Rd );   % KF gain 
IKC = eye(5) - K * Cd;
P_hat = IKC * P_prd * IKC' + K * Rd * K';      
x_hat = x_prd + K * (y - Cd * x_prd);          

% x = [ x^n y^n U chi omega_chi ]'
f = [ x_hat(3) * cos(x_hat(4))
      x_hat(3) * sin(x_hat(4))
     -alpha_1 * x_hat(3)
      x_hat(5)
     -alpha_2 * x_hat(5) ];

Ad = eye(5) + h_samp * ...
    [ 0 0 cos(x_hat(4)) -x_hat(3)*sin(x_hat(4)) 0
      0 0 sin(x_hat(4))  x_hat(3)*cos(x_hat(4)) 0
      0 0 -alpha_1 0 0
      0 0 0 0 1
      0 0 0 0 -alpha_2];
    
% Predictor (k+1)   
x_prd = x_hat + h_samp * f;
P_prd = Ad * P_hat * Ad' + Ed * Qd * Ed';

end

== matlab function mssSimulink/Marine craft models/Naval Postgraduate School AUV (npsAUV.m)/MATLAB Function ==
  data: x input; u input; xdot output; U output
function [xdot,U] = fcn(x,u)
% State vector: x = [ u v w p q r x y z phi theta psi ]' for
% an Autnomous Underwater Vehicle (AUV) at the Naval Postgraduate School.
% The length of the AUV is L = 5.3 m, while the state vector is defined as:
%
% u     = surge velocity          (m/s)
% v     = sway velocity           (m/s)
% w     = heave velocity          (m/s)
% p     = roll velocity           (rad/s)
% q     = pitch velocity          (rad/s)
% r     = yaw velocity            (rad/s)
% xpos  = position in x-direction (m)
% ypos  = position in y-direction (m)
% zpos  = position in z-direction (m)
% phi   = roll angle              (rad)
% theta = pitch angle             (rad)
% psi   = yaw angle               (rad)
%
% The input vector is :
%
% ui       = [ delta_r delta_s delta_b delta_bp delta_bs n ]'  where
%
% delta_r  = rudder angle                    (rad)
% delta_s  = port and starboard stern planes (rad)
% delta_b  = top and bottom bow planes       (rad)
% delta_bp = port bow plane                  (rad)
% delta_bs = starboard bow plane             (rad)
% n        = propeller shaft speed           (rpm)  
%
% Reference : Healey, A.J. and Lienard, D. (1993). Multivariable Sliding Mode Control 
%             for Autonomous Diving and Steering of Unmanned Underwater Vehicles,
%             IEEE Journal of Ocean Engineering, JOE-18(3):327-339

  [xdot,U] = npsauv(x,u);

end

== matlab function mssSimulink/Marine craft models/Otter USV (otter.m)/Otter USV ==
  settings: updateMethod=DISCRETE
  data: x input; n input; xdot output; mp input; rp input; V_c input; beta_c input; U output
function [xdot, U] = fcn(x,n,mp,rp,V_c,beta_c)

[xdot,U] = otter(x,n,mp,rp,V_c,beta_c);

end

== matlab function mssSimulink/Marine craft models/Deep submergence rescue vehicle (DSRV.m)/MATLAB Function ==
  data: x input; u input; xdot output; U output
function [xdot,U] = fcn(x,u)
% State vector:
%  w:       heave velocity                 (m/s)
%  q:       pitch velocity                 (rad/s)
%  x:       x-position                     (m)
%  z:       z-position, positive downwards (m)
%  theta:   pitch angle                    (rad)
%
% Input:
%  u:       delta (rad), where delta is the stern plane

[xdot,U] = DSRV(x,u);

end

== matlab function mssSimulink/Marine craft models/Mariner class cargo ship (mariner.m)/MATLAB Function ==
  data: x input; u input; xdot output; U output; U0 input
function [xdot,U] = fcn(x,u,U0)
% State vector: x = [ u v r x y psi delta ]'  for
% the Mariner class vessel L = 160.93 m, where
%  u     = pertubed surge velocity about Uo (m/s)
%  v     = pertubed sway velocity about zero (m/s)
%  r     = pertubed yaw velocity about zero (rad/s)
%  x     = position in x-direction (m)
%  y     = position in y-direction (m)
%  psi   = pertubed yaw angle about zero (rad)
%  delta = actual rudder angle (rad)
%
% The inputs are:
% 
%  u    = commanded rudder angle (rad)
%  U0   = nominal speed (optionally). Default value is U0 = 7.7175 m/s = 15 knots.
%
% Reference: M.S. Chislett and J. Stroem-Tejsen (1965). Planar Motion Mechanism Tests 
%            and Full-Scale Steering and Maneuvering Predictions for a Mariner Class Vessel,
%            Technical Report Hy-5, Hydro- and Aerodynamics Laboratory, Lyngby, Denmark.

 [xdot,U] = mariner(x,u,U0);

end

== matlab function mssSimulink/Marine craft models/Remus 100 AUV (remus100.m)/MATLAB Function ==
  data: x input; ui input; Vc input; xdot output; U output; betaVc input
function [xdot,U] = fcn(x,ui,Vc,betaVc)
% State vector: x = [ u v w p q r x y z phi theta psi ]' and speed U in m/s  
% (optionally) for the Remus 100 autonomous underwater vehicle (AUV). The 
% length of the AUV is L = 1.7 m, while the state vector is defined as:
%
%  u:       surge velocity          (m/s)
%  v:       sway velocity           (m/s)
%  w:       heave velocity          (m/s)
%  p:       roll rate               (rad/s)
%  q:       pitch rate              (rad/s)
%  r:       yaw rate                (rad/s)
%  x:       North position          (m)
%  y:       East position           (m)
%  z:       downwards position      (m)
%  phi:     roll angle              (rad)
%  theta:   pitch angle             (rad)
%  psi:     yaw angle               (rad)
%
% The control inputs are:
%
%  ui = [ delta_r delta_s n ]'  where
%
%    delta_r:   rudder angle (rad)
%    delta_s:   aft stern plane (rad) 
%    n:         propeller revolution (rpm)
%
% The last arguments Vc and betaVc are optional arguments for ocean current 
% speed and direction expressed in NED. 

  [xdot,U] = remus100(x,ui,Vc,betaVc);

end

== matlab function mssSimulink/Guidance/LOS guidance law for course autopilot ==
  settings: updateMethod=DISCRETE
  data: x input; y input; chi_ref output; Delta_h input; R_switch input; xdata input; ydata input
function chi_ref = fcn(x,y,Delta_h,R_switch,xdata,ydata)

% waypoints
wpt.pos.x = xdata;
wpt.pos.y = ydata;

chi_ref = LOSchi(x,y,Delta_h,R_switch,wpt);
    
end

== matlab function mssSimulink/Guidance/ILOS guidance law for heading autopilot ==
  settings: updateMethod=DISCRETE
  data: x input; y input; psi_ref output; Delta_h input; kappa input; R_switch input; xdata input; ydata input; h input
function psi_ref = fcn(x,y,Delta_h,kappa,R_switch,xdata,ydata,h)

% waypoints
wpt.pos.x = xdata;
wpt.pos.y = ydata;

% ILOS guidance law
psi_ref= ILOSpsi(x,y,Delta_h,kappa,h,R_switch,wpt);

end
